simulink model "commhdlQPSKTxRxLoopback"  (R2025b)
settings: Solver=FixedStepDiscrete  StartTime=0.0  StopTime=stopTime  RelTol=1e-3
PostLoadFcn:
  | hScopeConfig = get_param([gcs '/Receiver/QPSK Rx/Frequency and Time Synchronizer/Symbol Synchronizer/No HDL/QPSK Receiver Eye Diagram'],'ScopeConfiguration');
  | 
  | hScopeConfig.OpenAtSimulationStart = false;
  | hScopeConfig.Visible = false;
  | SamplesPerSymbol = 4;
  | %UpsamplesRx = 1;
  | clear hScopeConfig
InitFcn:
  | commhdlQPSKTxRxModelInit;
  | % Rate bridge: ADRV9002/Jupiter radio runs at 15.36 MHz = 2x the 7.68 MHz
  | % (4 samples/symbol @ Rsym=1.92 MHz) the QPSK Rx requires. The deployed
  | % Receiver must downsample the ADC stream by 2. UpsamplesRx=1 fed the QPSK
  | % Rx 8 sps (2x-upsampled) and broke symbol sync / the loopback bit check.
  | UpsamplesRx = 1;   %% T8 RATE FIX: rail 15.36e6 == ADC bus rate,
  | %% no ingress decimation (was 2 when the rail sat on the 7.68e6 rung)
  | UpsamplesTx = 1;
  | clear simTimingOffset;
StopFcn:
  | if exist('simTimingOffset','var')
  |   disp('Simulation completed');
  |   %QPSKTxRxVerification;
  | end
undefined symbols (not defined in the file or in its folder): Add, Config, fsym, randsrc, RandStream, Rsym, Shift
libraries: hdlsllib x141, simulink x43, dspsigops x34, dsphdlfiltering2 x6, dsphdlsigops2 x4, dsphdlmathfun2 x4, commdigbbndpm3 x4, dspmlti4 x2, commchan3 x1, commrflib2 x1, commcnvcod2 x1
(part 1 of 8)
CloseFcn:
  | clear Config CSLatency dataBits dataIn DBPP DescramblerLatency endLoc ...
  |         errSym errWaveform falsePacketsNo FCLatency idx initFramesNotToCompareInRx ...
  |         Nframes nReceivedBits PALatency PDLatency pktNo QPSKDemodLatency ...
  |         refQPSKSym refTxWaveform Rsym RxBits RxOut RxOutEnd RxOutSrt ...
  |         simAfterCS simBeforeSS simPeakFind simQPSKSym simSyncedPackets ...
  |         simTimingOffset simTxWaveform srtLoc SSLatency stopTime tout trueOffset ...
  |         TxBits validIn vPktNo
  | clear SamplesPerSymbol nErrBits nErrPkts nMissedPkts TxSymbolsMaxError TxWaveformMaxError
Description:
  | frame=f1536 variant=jupiter_240k5_byte(sps4/Rsym3840000-T8ratefix,K5[35 23]TB25 rx+GATED-txenc,ROMf1536+byteDMA,noscr+nodescr,taps 0x150/0x154/0x15C,agcEn10,txds 0x158,WPP191) pre=variant_pre_composite_verif+cfc_a12+bytek5 build=12-Aug-2026 10:18:16
settings Model: DataTypeOverride=Off  Creator=The MathWorks, Inc.  LastModifiedBy=tcollins
settings SolverCC: AlgebraicLoopSolver=TrustRegion  MaxZcPerStep=1.0
settings DataIOCC: ReturnWorkspaceOutputs=off
settings OptimizationCC: BlockReduction=off  ConditionallyExecuteInputs=off  DefaultParameterBehavior=Inlined  ReuseModelBlockBuffer=off
settings DebuggingCC: AlgebraicLoopMsg=error  SingleTaskRateTransMsg=error  UnconnectedInputMsg=warning  UnconnectedOutputMsg=warning  UnconnectedLineMsg=warning  SubsystemReferenceDiagnosticForUnitTest=warning
settings HardwareCC: ProdBitPerPointer=32.0  ProdBitPerSizeT=32.0  ProdBitPerPtrDiffT=32.0  ProdLargestAtomicFloat=None  ProdIntDivRoundTo=Undefined  ProdEndianess=Unspecified  ProdWordSize=32.0  ProdHWDeviceType=ASIC/FPGA->ASIC/FPGA  TargetBitPerLong=64.0  TargetBitPerPointer=64.0  TargetBitPerSizeT=64.0  TargetBitPerPtrDiffT=64.0  TargetLongLongMode=on  TargetIntDivRoundTo=Zero  TargetEndianess=LittleEndian  TargetWordSize=64.0  TargetHWDeviceType=Custom Processor->MATLAB Host Computer  ProdEqTarget=off
settings ModelReferenceCC: EnableRefExpFcnMdlSchedulingChecks=on
settings RTWCC: GPUComputeCapability=3.5  DLArmComputeVersion=19.05

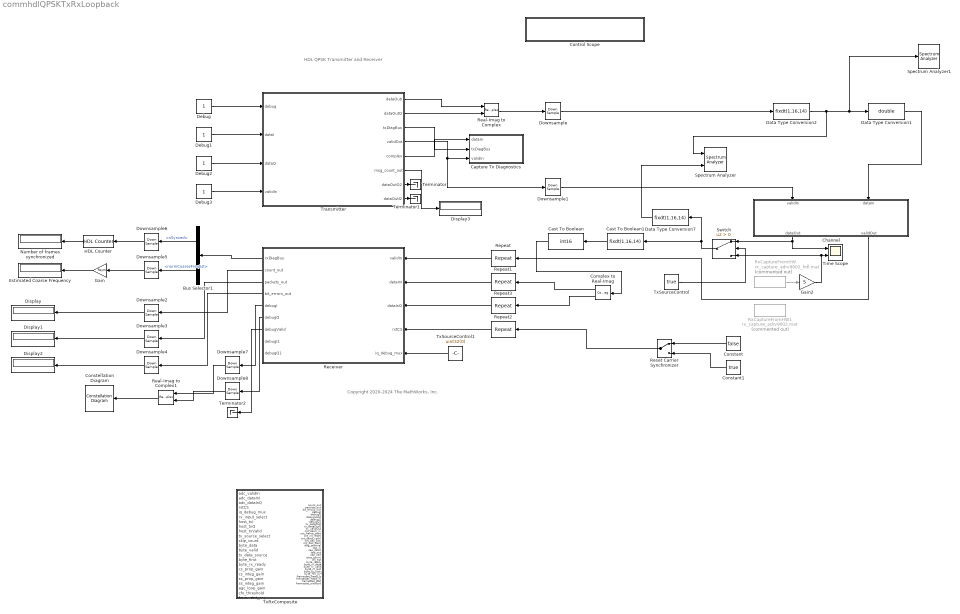
== system commhdlQPSKTxRxLoopback ==
  note: HDL QPSK Transmitter and Receiver
  note: Copyright 2020-2024 The MathWorks, Inc.
  Bus Selector1 : BusSelector  OutputSignals=nSynced,normCoarseFreqEst
  Capture Tx Diagnostics : Subsystem
  Cast To Boolean : DataTypeConversion  OutDataTypeStr=int16  ConvertRealWorld=Stored Integer (SI)  SaturateOnIntegerOverflow=off  RndMeth=Floor
  Cast To Boolean1 : DataTypeConversion  OutDataTypeStr=fixdt(1,16,14)  SaturateOnIntegerOverflow=off  RndMeth=Floor
  Channel : Subsystem  mask{EbN0dB=40, CFO=1e3, CPO=135, fractionalTimingOffset=0.55, timingFrequencyOffset=2}
      mask prompts: EbN0dB "Eb/N0 (in dB) :"; CFO "Carrier Frequency Offset (in Hz):"; CPO "Carrier Phase Offset (in Degrees) :"; fractionalTimingOffset "Fractional Timing Offset ( <1 ) :"; timingFrequencyOffset "Timing Frequency Offset (in PPM) :"
      mask init:
      | validateattributes(fractionalTimingOffset,{'double'},{'finite','scalar','nonnegative','>=',0,'<',1},'','fractionalTimingOffset');
      | validateattributes(timingFrequencyOffset,{'double'},{'finite','scalar','nonnegative'},'','timingFrequencyOffset');
      | validateattributes(EbN0dB,{'double'},{'scalar'},'','EbN0dB');
      | validateattributes(CFO,{'double'},{'finite','scalar',},'','CFO');
      | validateattributes(CPO,{'double'},{'finite','scalar'},'','CPO');
      | 
      | BitsPerSymbol = 2;      % QPSK
      | EbN0          = 10^(EbN0dB/10);
      | EsN0          = BitsPerSymbol*EbN0;
      | noiseVariance = 1/EsN0;  % QPSK symbol energy is normalized to 1 i.e. Es = 1
      | 
      | clear BitsPersymbol EbN0 EsN0
      settings: PortSchema="{\"entries\":[{\"content\":{\"sides\":[{\"content\":{\"connectorIds\":[]},\"type\":\"ConnectorPlacement.EquallySpacedRectSide\",\"uuid\":\"aa9ac445-3d73-401b-8e6c-a43fa6f53e3e\"},{\"content\":{\"connectorIds\":[],\"side\":\"RIGHT\"},\"type\":\"ConnectorPlacement.EquallySpacedRectSide\",\"uuid\":\"c8fbe2c1-ad18-4b81-8824-4fece19db9b5\"},{\"content\":{\"connectorIds\":[\"In1\",\"In2\"],\"side\":\"TOP\"},\"type\":\"ConnectorPlacement.EquallySpacedRectSide\",\"uuid\":\"2fdd8701-02b7-4a19-ab6e-54d2593732fa\"},{\"content\":{\"connectorIds\":[\"Out1\",\"Out2\"],\"side\":\"BOTTOM\"},\"type\":\"ConnectorPlacement.EquallySpacedRectSide\",\"uuid\":\"bd6ca111-71ba-47de-a918-1bcd41b09175\"}]},\"type\":\"ConnectorPlacement.EquallySpacedConnector\",\"uuid\":\"c410269f-5de3-4a8f-bc07-850237ff35fb\"}],\"packageUris\":[\"http://schema.mathworks.com/mf0/Connector/R2020b\"],\"version\":\"1.0\"}"
      mask DialogControl DescGroupVar Prompt: Channel
      mask Display: disp(['Double-Click' newline 'to set channel']);
  Complex to Real-Imag : ComplexToRealImag
  Constant : Constant  Value=false  SampleTime=1/(Rsym*Config.SamplesPerSymbol)
  Constant1 : Constant  Value=true  SampleTime=1/(Rsym*Config.SamplesPerSymbol)
  Constellation Diagram : ConstellationDiagram  WindowPosition=[594.000000,164.000000,600.000000,600.000000,]  Visible=on  ScopeFrameLocation=window  SymbolsToDisplaySource=Property  SymbolsToDisplay=1000  XLimits=[-1.375,8542.5]  YLimits=[-1.375,8542.5]  AxesLimits=[-1.375,8542.5]  MaximizeAxes=on  DefaultConfigurationName=comm.scopes.ConstellationDiagramBlockCfg
  Control Scope : Subsystem
      settings: OpenFcn=|
      | hScopeConfig1 = get_param([gcs '/Capture Tx Diagnostics/QPSK Transmitter Constellations'],'ScopeConfiguration');
      | hScopeConfig2 = get_param([gcs '/QPSK Rx/Frequency and Time Synchronizer/Symbol Synchronizer/No HDL/QPSK Receiver Eye Diagram'],'ScopeConfiguration');
      | hScopeConfig3 = get_param([gcs '/QPSK Rx/Frequency and Time Synchronizer/Symbol Synchronizer/No HDL/No HDL/QPSK Receiver Constellation 1'],'ScopeConfiguration');
      | hScopeConfig4 = get_param([gcs '/QPSK Rx/Frequency and Time Synchronizer/No HDL/QPSK Receiver Constellations 2'],'ScopeConfiguration');
      | hScopeConfig5 = get_param([gcs '/QPSK Rx/Frequency and Time Synchronizer/Preamble Detector/No HDL/Correlation Time Scope'],'ScopeConfiguration');
      | 
      | 
      | 
      | if all([hScopeConfig1.Visible hScopeConfig2.Visible hScopeConfig3.Visible hScopeConfig4.Visible hScopeConfig5.Visible])
      |    hScopeConfig1.Visible = false;
      |    hScopeConfig2.Visible = false;
      |    hScopeConfig3.Visible = false;
      |    hScopeConfig4.Visible = false;
      |    hScopeConfig5.Visible = false;
      | else
      |    hScopeConfig1.Visible = true;
      |    hScopeConfig2.Visible = true;
      |    hScopeConfig3.Visible = true;
      |    hScopeConfig4.Visible = true;
      |    hScopeConfig5.Visible = true;
      | end
      | 
      | clear hScopeConfig1 hScopeConfig2 hScopeConfig3 hScopeConfig4 hScopeConfig5;
      mask Display: disp('Double-click to turn on/off the Scopes');
  Data Type Conversion1 : DataTypeConversion  OutDataTypeStr=double  SaturateOnIntegerOverflow=off  RndMeth=Floor
  Data Type Conversion2 : DataTypeConversion  OutDataTypeStr=fixdt(1,16,14)  ConvertRealWorld=Stored Integer (SI)  SaturateOnIntegerOverflow=off  RndMeth=Floor
  Data Type Conversion7 : DataTypeConversion  OutDataTypeStr=fixdt(1,16,14)  SaturateOnIntegerOverflow=off  RndMeth=Floor
  Debug : Constant  OutDataTypeStr=uint32  SampleTime=-1
  Debug1 : Constant  OutDataTypeStr=int16  SampleTime=-1
  Debug2 : Constant  OutDataTypeStr=int16  SampleTime=-1
  Debug3 : Constant  OutDataTypeStr=boolean  SampleTime=-1
  Display{,1..3} (4 alike) : Display
  Downsample : DownSample  N=UpsamplesTx  RateOptions=Allow multirate processing
  Downsample1 : DownSample  N=UpsamplesTx  RateOptions=Allow multirate processing
  Downsample{2..8} (7 alike) : DownSample  N=UpsamplesRx  RateOptions=Allow multirate processing
  Estimated Coarse Frequency : Display
  Gain : Gain  Gain=Rsym
  Gain2 : Gain  Gain=5
  HDL Counter : hdlsllib/Sources/HDL Counter  CountType=Free running  CountInit=0  CountStep=1  CountMax=25  CountFromType=Initial value  CountFrom=0  CountResetPort=off  CountLoadPort=off  CountEnbPort=on  CountDirPort=off  CountHitOutputPort=off  CountDataType=Unsigned  CountWordLen=32  CountFracLen=0  CountSampTime=1
  Number of frames synchronized : Display
  Real-Imag to Complex : RealImagToComplex
  Real-Imag to Complex1 : RealImagToComplex
  Receiver : Subsystem  TreatAsAtomicUnit=on
  Repeat{,1..3} (4 alike) : dspsigops/Repeat  FactorSource=Dialog parameter  N=UpsamplesRx  Nmax=16  InputProcessing=Columns as channels (frame based)  RateOptions=Allow multirate processing  ic=0  mode=Unused parameter value
      settings: LibrarySourceBlock=commsequence2/Repeat
  Reset Carrier Synchronizer : ManualSwitch
  RxCaptureFromHW : FromFile  Commented=on  FileName=rx_capture_adrv9002_hdl.mat  OutDataTypeStr=double  SampleTime=1/(Rsym*Config.SamplesPerSymbol)  ExtrapolationBeforeFirstDataPoint=Hold first value  InterpolationWithinTimeRange=Zero order hold  ExtrapolationAfterLastDataPoint=Hold last value
  RxCaptureFromHW1 : FromFile  Commented=on  FileName=rx_capture_adrv9002.mat  OutDataTypeStr=double  SampleTime=1/(Rsym*Config.SamplesPerSymbol)  ExtrapolationBeforeFirstDataPoint=Hold first value  InterpolationWithinTimeRange=Zero order hold  ExtrapolationAfterLastDataPoint=Hold last value
  Spectrum Analyzer : SpectrumAnalyzer  NumInputPorts=2  WindowPosition=[494.000000,214.000000,800.000000,500.000000,]  Visible=on  ScopeFrameLocation=window  WindowInvariantSamplesPerUpdate=on  Span=7680000  StartFrequency=-3840000  StopFrequency=3840000  YLimits=[-47.9968 8.4452]
  Spectrum Analyzer1 : SpectrumAnalyzer  WindowPosition=[494.000000,214.000000,800.000000,500.000000,]  Visible=on  ScopeFrameLocation=window  WindowInvariantSamplesPerUpdate=on  Span=7680000  StartFrequency=-3840000  StopFrequency=3840000  YLimits=[-71.5508 10.9276]
  Switch : Switch  Criteria=u2 > Threshold  SaturateOnIntegerOverflow=off  InputSameDT=off
  Terminator : Terminator
  Terminator1 : Terminator
  Terminator2 : Terminator
  Time Scope : Scope  NumInputPorts=2
      settings: TimeUnits=Metric (based on Time Span)  ActiveDisplayYMinimum=-1.0052287666621835  ActiveDisplayYMaximum=0.87958747263253323  YLabel=Amplitude
  Transmitter : Subsystem  TreatAsAtomicUnit=on
  TxRxComposite : Subsystem
  TxSourceControl : Constant  Value=true  SampleTime=-1
  TxSourceControl1 : Constant  Value=uint32(0)  SampleTime=-1
  wires:
  Bus Selector1/1 -> Downsample6/1  "<nSynced>"
  HDL Counter/1 -> Number of frames synchronized/1
  Bus Selector1/2 -> Downsample5/1  "<normCoarseFreqEst>"
  Gain/1 -> Estimated Coarse Frequency/1
  Data Type Conversion1/1 -> Channel/2(dataIn)
  Constant/1 -> Reset Carrier Synchronizer/1
  Constant1/1 -> Reset Carrier Synchronizer/2
  Channel/1(dataOut) -> Time Scope/1, Switch/1
  Switch/1 -> Data Type Conversion7/1, Cast To Boolean1/1
  TxSourceControl/1 -> Switch/2
  RxCaptureFromHW/1 -> Gain2/1
  Gain2/1 -> Switch/3, Time Scope/2
  Transmitter/4(validOut) -> Downsample1/1, Capture Tx Diagnostics/3(validIn)
  Transmitter/3(txDiagBus) -> Capture Tx Diagnostics/2(txDiagBus)
  Debug/1 -> Transmitter/1(debug)
  Channel/2(validOut) -> Repeat/1
  Reset Carrier Synchronizer/1 -> Repeat2/1
  Receiver/2(count_out) -> Downsample2/1
  Receiver/3(packets_out) -> Downsample3/1
  Receiver/4(bit_errors_out) -> Downsample4/1
  Debug2/1 -> Transmitter/3(dataQ)
  Debug1/1 -> Transmitter/2(dataI)
  Debug3/1 -> Transmitter/4(validIn)
  Transmitter/1(dataOutI) -> Real-Imag to Complex/1
  Transmitter/2(dataOutQ) -> Real-Imag to Complex/2
  Real-Imag to Complex/1 -> Downsample/1
  Transmitter/5(complex) -> Capture Tx Diagnostics/1(dataIn)
  Data Type Conversion2/1 -> Spectrum Analyzer/1, Spectrum Analyzer1/1, Data Type Conversion1/1
  Transmitter/6(msg_count_out) -> Display3/1
  Downsample/1 -> Data Type Conversion2/1
  Downsample1/1 -> Channel/1(validIn)
  Repeat/1 -> Receiver/1(validIn)
  Repeat1/1 -> Receiver/2(dataInI)
  Repeat2/1 -> Receiver/4(rstCS)
  Downsample2/1 -> Display/1
  Downsample3/1 -> Display1/1
  Downsample4/1 -> Display2/1
  Receiver/1(rxDiagBus) -> Bus Selector1/1
  Downsample5/1 -> Gain/1
  Downsample6/1 -> HDL Counter/1
  Transmitter/7(dataOutQ2) -> Terminator/1
  Transmitter/8(dataOutI2) -> Terminator1/1
  TxSourceControl1/1 -> Receiver/5(iq_debug_mux)
  Complex to Real-Imag/1 -> Repeat1/1
  Complex to Real-Imag/2 -> Repeat3/1
  Data Type Conversion7/1 -> Spectrum Analyzer/2
  Cast To Boolean/1 -> Complex to Real-Imag/1
  Repeat3/1 -> Receiver/3(dataInQ)
  Cast To Boolean1/1 -> Cast To Boolean/1
  Receiver/5(debugI) -> Downsample7/1
  Receiver/6(debugQ) -> Downsample8/1
  Downsample7/1 -> Real-Imag to Complex1/1
  Downsample8/1 -> Real-Imag to Complex1/2
  Real-Imag to Complex1/1 -> Constellation Diagram/1
  Receiver/7(debugValid) -> Terminator2/1

== system commhdlQPSKTxRxLoopback/Capture Tx Diagnostics ==
  dataIn : Inport
  txDiagBus : Inport  Port=2
  validIn : Inport  Port=3
  Bus Selector : BusSelector  OutputSignals=QPSKConstellationPoints,QPSKConstellationValid
  Data Type Conversion : DataTypeConversion  OutDataTypeStr=double  SaturateOnIntegerOverflow=off  RndMeth=Floor
  Data Type Conversion1 : DataTypeConversion  OutDataTypeStr=double  SaturateOnIntegerOverflow=off  RndMeth=Floor
  QPSK Transmitter Constellations : ConstellationDiagram  NumInputPorts=2  WindowPosition=[708.000000,285.000000,372.000000,357.000000,]  Visible=on  ScopeFrameLocation=window  SymbolsToDisplaySource=Property  SymbolsToDisplay=10000  ReferenceConstellation="{[0.70711+0.70711i        -0.70711+0.70711i        -0.70711-0.70711i         0.70711-0.70711i],[0.70711+0.70711i        -0.70711+0.70711i        -0.70711-0.70711i         0.70711-0.70711i]}"  ReferenceMarker={''o'',''o''}  ReferenceColor={[1 0 0],[1 0 0]}  XLimits=[-0.94638 0.94638]  YLimits=[-0.94638 0.94638]  AxesLimits=[-0.94638 0.94638]  ShowLegend=on  DefaultConfigurationName=comm.scopes.ConstellationDiagramBlockCfg
      settings: OpenAtSimulationStart=off
  Subsystem : Subsystem
  Subsystem1 : Subsystem
  Unit Delay Enabled Synchronous : hdlsllib/Discrete/Unit Delay Enabled Synchronous  InitialCondition=0.0  SampleTime=-1
  Unit Delay Enabled Synchronous1 : hdlsllib/Discrete/Unit Delay Enabled Synchronous  InitialCondition=0.0  SampleTime=-1
  wires:
  txDiagBus/1 -> Bus Selector/1
  Bus Selector/1 -> Data Type Conversion/1  "<QPSKConstellationPoints>"
  Data Type Conversion/1 -> Unit Delay Enabled Synchronous/1, Subsystem/1(In1)
  dataIn/1 -> Data Type Conversion1/1
  Bus Selector/2 -> Subsystem/Enable, Unit Delay Enabled Synchronous/2  "<QPSKConstellationValid>"
  Data Type Conversion1/1 -> Unit Delay Enabled Synchronous1/1, Subsystem1/1(In1)
  validIn/1 -> Subsystem1/Enable, Unit Delay Enabled Synchronous1/2
  Unit Delay Enabled Synchronous1/1 -> QPSK Transmitter Constellations/2  "RRC Filtered Output"
  Unit Delay Enabled Synchronous/1 -> QPSK Transmitter Constellations/1  "Modulator Output"

== system commhdlQPSKTxRxLoopback/Channel ==
  validIn : Inport
  dataIn : Inport  Port=2
  AWGN Channel : commchan3/AWGN Channel  LegacyMode=on  NoiseMethod="Signal to noise ratio  (SNR)"  noiseMode=Variance from mask  EbNo=EbN0dB  EsNo=10  SNR=10  BitsPerSymbol=2  SignalPower=1  SpecifySymbolPeriod=off  SamplesPerSymbol=1  SymbolPeriod=1/fsym  VarianceSource=Parameter  Variance=noiseVariance  RandomStream=Global stream  Seed=67  SimulateUsing=Code generation
  Add : Sum  Inputs=|++
  Add1 : Sum  Inputs=++|
  Constant : Constant  Value=fractionalTimingOffset  SampleTime=-1
  Constant1 : Constant  Value=timingFrequencyOffset * 1e-6  SampleTime=-1
  Delay : Delay  DelayLength=1
  Mod 1 : Subsystem
  Phase/ Frequency Offset : commrflib2/Phase// Frequency Offset  phaseOffset=CPO  freqPort=off  freqOffset=CFO
  Variable Fractional Delay : dspsigops/Variable Fractional Delay  mode=OBSOLETE  modeActive=Linear  L=4  FarrowL=4  R=10  alpha=1  dmax=100  InputProcessing=Columns as channels (frame based)  ic=0  noDFT=off  fallbackFIR=Clip to the minimum value necessary for centered kernel  fallbackFarrow=Clip to the minimum value necessary for centered kernel  roundingMode=Zero  overflowMode=off
  dataOut : Outport
  validOut : Outport  Port=2
  wires:
  AWGN Channel/1 -> Phase/ Frequency Offset/1
  Variable Fractional Delay/1 -> AWGN Channel/1
  dataIn/1 -> Variable Fractional Delay/1
  Constant1/1 -> Add/1
  Delay/1 -> Add/2, Add1/2
  Add/1 -> Delay/1
  Add1/1 -> Mod 1/1(In1)
  Constant/1 -> Add1/1
  Mod 1/1(Out1) -> Variable Fractional Delay/2
  Phase/ Frequency Offset/1 -> dataOut/1
  validIn/1 -> validOut/1

== system commhdlQPSKTxRxLoopback/Control Scope ==

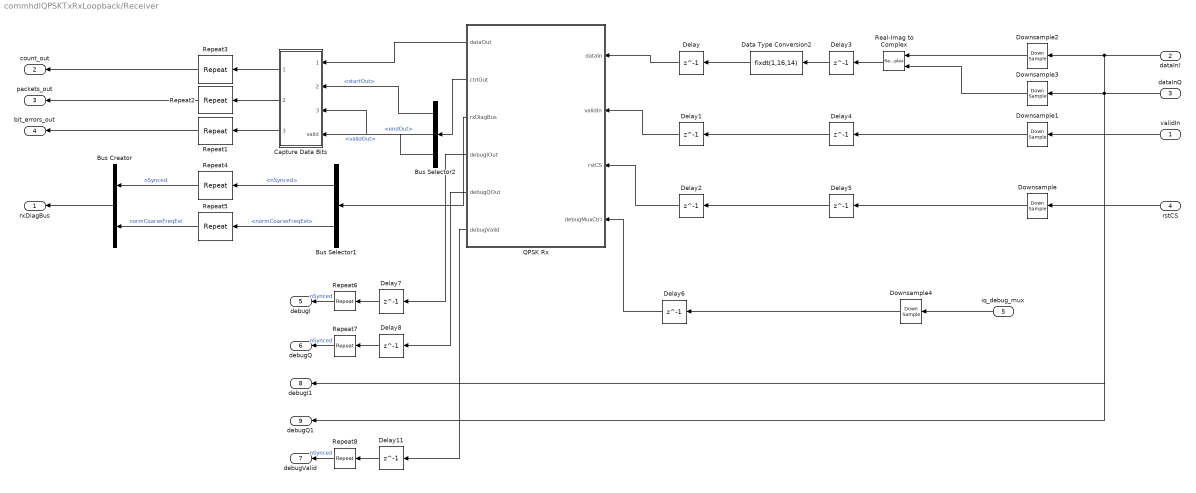
== system commhdlQPSKTxRxLoopback/Receiver ==
  validIn : Inport
  dataInI : Inport  Port=2
  dataInQ : Inport  Port=3
  rstCS : Inport  Port=4
  iq_debug_mux : Inport  Port=5  OutDataTypeStr=uint32
  Bus Creator : BusCreator  Inputs=2
  Bus Selector1 : BusSelector  OutputSignals=nSynced,normCoarseFreqEst
  Bus Selector2 : BusSelector  OutputSignals=startOut,endOut,validOut
  Capture Data Bits : Subsystem
  Data Type Conversion2 : DataTypeConversion  OutDataTypeStr=fixdt(1,16,14)  ConvertRealWorld=Stored Integer (SI)  SaturateOnIntegerOverflow=off  RndMeth=Floor
  Delay{,1..8,11} (10 alike) : Delay  DelayLength=1
  Downsample{,1..4} (5 alike) : DownSample  N=UpsamplesRx  RateOptions=Allow multirate processing
  QPSK Rx : Subsystem
      mask init:
      | integAvgLen = 2^12;
      | 
      | RxParams            = commhdlQPSKTxRxParameters();
      | Preamble            = RxParams.Preamble;
      | QPSKConstellation   = RxParams.QPSKConstellation;
      | dataBitsPerPacket   = RxParams.DataBitsPerPacket;
      | SamplesPerSymbol    = RxParams.SamplesPerSymbol;
      | RRCCoef             = RxParams.RRCCoef;
      | bitsPerPacket        = RxParams.BitsPerPacket;
      | 
      | rxPreambleMFCoeffs  = RxParams.rxPreambleMFCoeffs;
      | preambleSymbols     = RxParams.preambleSymbols;
      | ThresoldGainFac     = RxParams.ThresoldGainFac;
      | 
      | % AGC Parameters
      | AGCReference           = RxParams.AGCReference;
      | AGCLoopGain            = RxParams.AGCLoopGain;
      | 
      | % CS parameters
      | CSKp                   = RxParams.CSKp;
      | CSK0                   = RxParams.CSK0;  
      | CSLoopFilterPropGain   = RxParams.CSLoopFilterPropGain;
      | CSLoopFilterIntegGain  = RxParams.CSLoopFilterIntegGain;
      | CFOChangeDetectThreshold = RxParams.CFOChangeDetectThreshold;
      | 
      | % SS parameters
      | SSKp                   = RxParams.SSKp; 
      | SSK0                   = RxParams.SSK0;  
      | SSLoopFilterPropGain   = RxParams.SSLoopFilterPropGain;
      | SSLoopFilterIntegGain  = RxParams.SSLoopFilterIntegGain;
      | 
      | % preamble detector parameters
      | searchSamples          = RxParams.SearchSamples;
      | 
      | clear RxParams;
  Real-Imag to Complex : RealImagToComplex
  Repeat{1..8} (8 alike) : dspsigops/Repeat  FactorSource=Dialog parameter  N=UpsamplesRx  Nmax=16  InputProcessing=Columns as channels (frame based)  RateOptions=Allow multirate processing  ic=0  mode=Unused parameter value
      settings: LibrarySourceBlock=commsequence2/Repeat
  rxDiagBus : Outport
  count_out : Outport  Port=2
  packets_out : Outport  Port=3
  bit_errors_out : Outport  Port=4
  debugI : Outport  Port=5
  debugQ : Outport  Port=6
  debugValid : Outport  Port=7
  debugI1 : Outport  Port=8
  debugQ1 : Outport  Port=9
  wires:
  Bus Selector2/1 -> Capture Data Bits/2(dataSrt)  "<startOut>"
  QPSK Rx/1(dataOut) -> Capture Data Bits/1(dataOut)
  QPSK Rx/2(ctrlOut) -> Bus Selector2/1
  Bus Selector2/2 -> Capture Data Bits/3(dataEnd)  "<endOut>"
  rstCS/1 -> Downsample/1
  validIn/1 -> Downsample1/1
  Bus Selector2/3 -> Capture Data Bits/4(valid)  "<validOut>"
  Capture Data Bits/1(count_out) -> Repeat3/1
  Capture Data Bits/2(packets_out) -> Repeat2/1
  Capture Data Bits/3(bit_errors_out) -> Repeat1/1
  Downsample1/1 -> Delay4/1
  Repeat1/1 -> bit_errors_out/1
  Repeat2/1 -> packets_out/1
  Repeat3/1 -> count_out/1
  QPSK Rx/3(rxDiagBus) -> Bus Selector1/1
  Bus Creator/1 -> rxDiagBus/1
  Bus Selector1/1 -> Repeat4/1  "<nSynced>"
  Bus Selector1/2 -> Repeat5/1  "<normCoarseFreqEst>"
  Repeat4/1 -> Bus Creator/1  "nSynced"
  Repeat5/1 -> Bus Creator/2  "normCoarseFreqEst"
  dataInQ/1 -> debugQ1/1, Downsample3/1
  dataInI/1 -> debugI1/1, Downsample2/1
  Real-Imag to Complex/1 -> Delay3/1
  Downsample2/1 -> Real-Imag to Complex/1
  Downsample3/1 -> Real-Imag to Complex/2
  Data Type Conversion2/1 -> Delay/1
  Delay/1 -> QPSK Rx/1(dataIn)
  Delay1/1 -> QPSK Rx/2(validIn)
  Delay2/1 -> QPSK Rx/3(rstCS)
  Delay3/1 -> Data Type Conversion2/1
  Delay4/1 -> Delay1/1
  Delay5/1 -> Delay2/1
  QPSK Rx/4(debugIOut) -> Delay7/1
  QPSK Rx/5(debugQOut) -> Delay8/1
  Repeat6/1 -> debugI/1  "nSynced"
  Repeat7/1 -> debugQ/1  "nSynced"
  iq_debug_mux/1 -> Downsample4/1
  Delay6/1 -> QPSK Rx/4(debugMuxCtrl)
  Downsample4/1 -> Delay6/1
  Repeat8/1 -> debugValid/1  "nSynced"
  QPSK Rx/6(debugValid) -> Delay11/1
  Delay7/1 -> Repeat6/1
  Delay8/1 -> Repeat7/1
  Delay11/1 -> Repeat8/1
  Downsample/1 -> Delay5/1

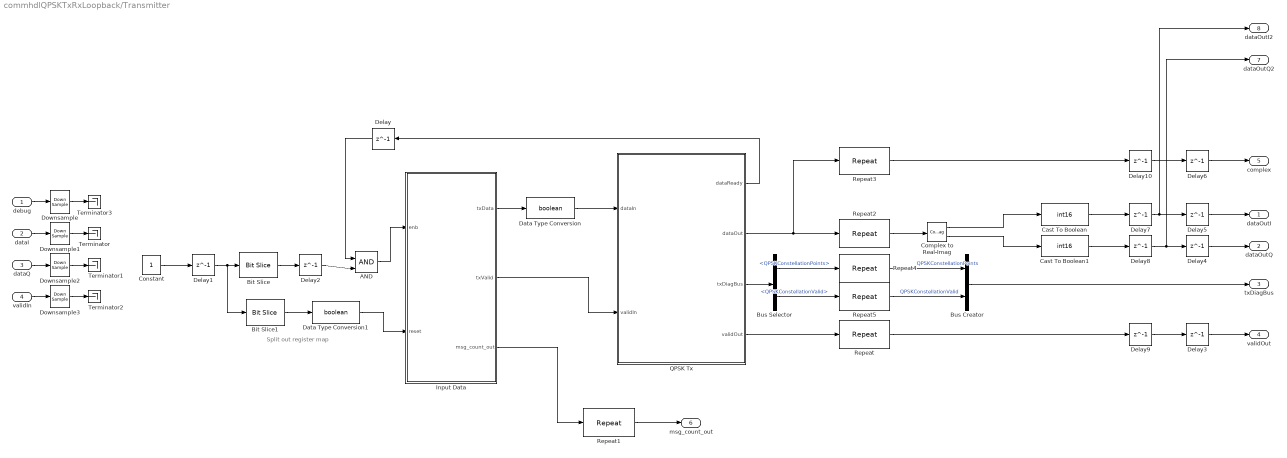
== system commhdlQPSKTxRxLoopback/Transmitter ==
  note: Split out register map
  debug : Inport  PortDimensions=1
  dataI : Inport  Port=2
  dataQ : Inport  Port=3
  validIn : Inport  Port=4
  AND : Logic  IconShape=distinctive  AllPortsSameDT=off  OutDataTypeStr=boolean
  Bit Slice : hdlsllib/Logic and Bit Operations/Bit Slice  lidx=0  ridx=0
  Bit Slice1 : hdlsllib/Logic and Bit Operations/Bit Slice  lidx=1  ridx=1
  Bus Creator : BusCreator  Inputs=2
  Bus Selector : BusSelector  OutputSignals=QPSKConstellationPoints,QPSKConstellationValid
  Cast To Boolean : DataTypeConversion  OutDataTypeStr=int16  ConvertRealWorld=Stored Integer (SI)  SaturateOnIntegerOverflow=off  RndMeth=Floor
  Cast To Boolean1 : DataTypeConversion  OutDataTypeStr=int16  ConvertRealWorld=Stored Integer (SI)  SaturateOnIntegerOverflow=off  RndMeth=Floor
  Complex to Real-Imag : ComplexToRealImag
  Constant : Constant  OutDataTypeStr=uint32  SampleTime=-1
  Data Type Conversion : DataTypeConversion  OutDataTypeStr=boolean  SaturateOnIntegerOverflow=off  RndMeth=Floor
  Data Type Conversion1 : DataTypeConversion  OutDataTypeStr=boolean  SaturateOnIntegerOverflow=off  RndMeth=Floor
  Delay{,1..10} (11 alike) : Delay  DelayLength=1
  Downsample{,1..3} (4 alike) : DownSample  N=UpsamplesTx  RateOptions=Allow multirate processing
  Input Data : Subsystem  mask{dataBits=reshape(repmat(randsrc(2240*1,1,[0,1],RandStream('mcg16807','Seed',0)), 59,1), [2240*59,1]), Rsym=3.84e6}
      mask prompts: dataBits "Data Bits :"; Rsym "Symbol Rate (in baud rate)  :"
      mask Display: disp(['Double-Click' newline 'to set data bits']);
  QPSK Tx : Subsystem
      mask init:
      | TxParams           = commhdlQPSKTxRxParameters();
      | Preamble            = TxParams.Preamble;
      | QPSKConstellation   = TxParams.QPSKConstellation;
      | dataBitsPerPacket   = TxParams.DataBitsPerPacket;
      | SamplesPerSymbol    = TxParams.SamplesPerSymbol;
      | RRCCoef             = TxParams.RRCCoef;
      | dataRAMAddrWidth    = TxParams.txDataRAMAddrWidth;
      | bitsPerPacket       = TxParams.BitsPerPacket;
      | 
      | clear TxParams;
  Repeat{,1..5} (6 alike) : dspsigops/Repeat  FactorSource=Dialog parameter  N=UpsamplesTx  Nmax=16  InputProcessing=Columns as channels (frame based)  RateOptions=Allow multirate processing  ic=0  mode=Unused parameter value
      settings: LibrarySourceBlock=commsequence2/Repeat
  Terminator{,1..3} (4 alike) : Terminator
  dataOutI : Outport
  dataOutQ : Outport  Port=2
  txDiagBus : Outport  Port=3
  validOut : Outport  Port=4
  complex : Outport  Port=5
  msg_count_out : Outport  Port=6
  dataOutQ2 : Outport  Port=7
  dataOutI2 : Outport  Port=8
  wires:
  Input Data/2(txValid) -> QPSK Tx/2(validIn)
  Input Data/1(txData) -> Data Type Conversion/1
  Data Type Conversion/1 -> QPSK Tx/1(dataIn)
  QPSK Tx/4(validOut) -> Repeat/1
  QPSK Tx/1(dataReady) -> Delay/1
  AND/1 -> Input Data/1(enb)
  Bit Slice/1 -> Delay2/1
  Delay/1 -> AND/1
  Delay1/1 -> Bit Slice1/1, Bit Slice/1
  Delay2/1 -> AND/2
  Bit Slice1/1 -> Data Type Conversion1/1
  Data Type Conversion1/1 -> Input Data/2(reset)
  dataI/1 -> Downsample1/1
  dataQ/1 -> Downsample2/1
  validIn/1 -> Downsample3/1
  Constant/1 -> Delay1/1
  debug/1 -> Downsample/1
  QPSK Tx/2(dataOut) -> Repeat3/1, Repeat2/1
  Complex to Real-Imag/1 -> Cast To Boolean/1
  Complex to Real-Imag/2 -> Cast To Boolean1/1
  Input Data/3(msg_count_out) -> Repeat1/1
  Repeat/1 -> Delay9/1
  Repeat2/1 -> Complex to Real-Imag/1
  Repeat3/1 -> Delay10/1
  Downsample/1 -> Terminator3/1
  Downsample1/1 -> Terminator/1
  Downsample2/1 -> Terminator1/1
  Downsample3/1 -> Terminator2/1
  Repeat1/1 -> msg_count_out/1
  QPSK Tx/3(txDiagBus) -> Bus Selector/1
  Bus Selector/1 -> Repeat4/1  "<QPSKConstellationPoints>"
  Repeat4/1 -> Bus Creator/1  "QPSKConstellationPoints"
  Bus Selector/2 -> Repeat5/1  "<QPSKConstellationValid>"
  Repeat5/1 -> Bus Creator/2  "QPSKConstellationValid"
  Bus Creator/1 -> txDiagBus/1
  Cast To Boolean/1 -> Delay7/1
  Cast To Boolean1/1 -> Delay8/1
  Delay3/1 -> validOut/1
  Delay4/1 -> dataOutQ/1
  Delay5/1 -> dataOutI/1
  Delay6/1 -> complex/1
  Delay7/1 -> dataOutI2/1, Delay5/1
  Delay8/1 -> dataOutQ2/1, Delay4/1
  Delay9/1 -> Delay3/1
  Delay10/1 -> Delay6/1

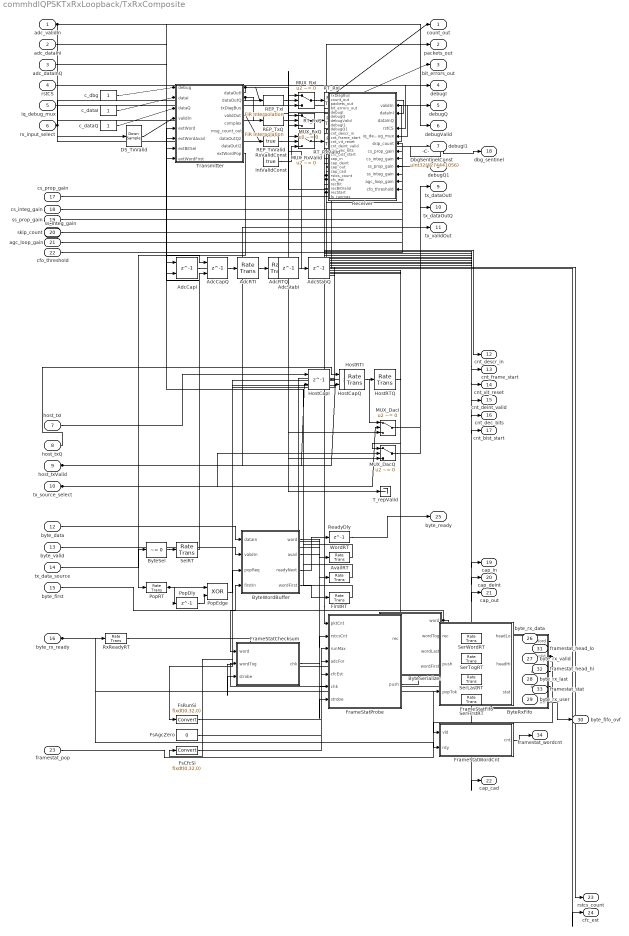
== system commhdlQPSKTxRxLoopback/TxRxComposite ==
  adc_validIn : Inport  OutDataTypeStr=boolean  SampleTime=1/30.72e6
  adc_dataInI : Inport  Port=2  OutDataTypeStr=int16  SampleTime=1/30.72e6
  adc_dataInQ : Inport  Port=3  OutDataTypeStr=int16  SampleTime=1/30.72e6
  rstCS : Inport  Port=4  OutDataTypeStr=boolean  SampleTime=1/15.36e6
  iq_debug_mux : Inport  Port=5  OutDataTypeStr=uint32  SampleTime=1/15.36e6
  rx_input_select : Inport  Port=6  OutDataTypeStr=boolean  SampleTime=1/15.36e6
  host_txI : Inport  Port=7  OutDataTypeStr=int16  SampleTime=1/30.72e6
  host_txQ : Inport  Port=8  OutDataTypeStr=int16  SampleTime=1/30.72e6
  host_txValid : Inport  Port=9  OutDataTypeStr=boolean  SampleTime=1/30.72e6
  tx_source_select : Inport  Port=10  OutDataTypeStr=uint32  SampleTime=1/15.36e6
  skip_count : Inport  Port=11  OutDataTypeStr=uint32  SampleTime=1/15.36e6
  byte_data : Inport  Port=12  OutDataTypeStr=uint64  SampleTime=1/30.72e6
  byte_valid : Inport  Port=13  OutDataTypeStr=boolean  SampleTime=1/30.72e6
  tx_data_source : Inport  Port=14  OutDataTypeStr=uint32  SampleTime=1/15.36e6
  byte_first : Inport  Port=15  OutDataTypeStr=boolean  SampleTime=1/30.72e6
  byte_rx_ready : Inport  Port=16  OutDataTypeStr=boolean  SampleTime=1/30.72e6
  cs_prop_gain : Inport  Port=17  OutDataTypeStr=uint32  SampleTime=1/15.36e6
  cs_integ_gain : Inport  Port=18  OutDataTypeStr=uint32  SampleTime=1/15.36e6
  ss_prop_gain : Inport  Port=19  OutDataTypeStr=uint32  SampleTime=1/15.36e6
  ss_integ_gain : Inport  Port=20  OutDataTypeStr=uint32  SampleTime=1/15.36e6
  agc_loop_gain : Inport  Port=21  OutDataTypeStr=uint32  SampleTime=1/15.36e6
  cfo_threshold : Inport  Port=22  OutDataTypeStr=uint32  SampleTime=1/15.36e6
  framestat_pop : Inport  Port=23  OutDataTypeStr=uint32  SampleTime=1/15.36e6
  AdcCapI : Delay  DelayLength=1  ShowEnablePort=on
      settings: InputPortMap=u0,e6
  AdcCapQ : Delay  DelayLength=1  ShowEnablePort=on
      settings: InputPortMap=u0,e6
  AdcRTI : RateTransition  OutPortSampleTime=1/15.36e6
  AdcRTQ : RateTransition  OutPortSampleTime=1/15.36e6
  AdcStabI : Delay  DelayLength=1
  AdcStabQ : Delay  DelayLength=1
  AvailRT : RateTransition  OutPortSampleTime=1/15.36e6
  ByteRxFifo : MATLAB Function  TreatAsAtomicUnit=on
  ByteSel : simulink/Logic and Bit Operations/Compare To Constant  relop=~=  const=0  OutDataTypeStr=boolean
  ByteSerializer : MATLAB Function  TreatAsAtomicUnit=on
  ByteWordBuffer : MATLAB Function  TreatAsAtomicUnit=on
  DS_TxValid : DownSample  N=1  RateOptions=Allow multirate processing  AllowArbitraryFixedInput=on
  DbgSentinelConst : Constant  Value=uint32(4274441056)  OutDataTypeStr=uint32  SampleTime=1/15.36e6
  FirstRT : RateTransition  OutPortSampleTime=1/15.36e6
  FrameStatChecksum : MATLAB Function  TreatAsAtomicUnit=on
  FrameStatFifo : MATLAB Function  TreatAsAtomicUnit=on
  FrameStatProbe : MATLAB Function  TreatAsAtomicUnit=on
  FrameStatWordCnt : MATLAB Function  TreatAsAtomicUnit=on
  FsAgcZero : Constant  Value=0  OutDataTypeStr=uint32
  FsCfcSi : DataTypeConversion  OutDataTypeStr=fixdt(0,32,0)  ConvertRealWorld=Stored Integer (SI)  SaturateOnIntegerOverflow=off  RndMeth=Floor
  FsRunSi : DataTypeConversion  OutDataTypeStr=fixdt(0,32,0)  ConvertRealWorld=Stored Integer (SI)  SaturateOnIntegerOverflow=off  RndMeth=Floor
  HostCapI : Delay  DelayLength=1  ShowEnablePort=on
      settings: InputPortMap=u0,e6
  HostCapQ : Delay  DelayLength=1  ShowEnablePort=on
      settings: InputPortMap=u0,e6
  HostRTI : RateTransition  OutPortSampleTime=1/30.72e6
  HostRTQ : RateTransition  OutPortSampleTime=1/30.72e6
  IntValidConst : Constant  Value=true  OutDataTypeStr=boolean  SampleTime=1/15.36e6
  MUX_DacI : Switch  Criteria=u2 ~= 0
  MUX_DacQ : Switch  Criteria=u2 ~= 0
  MUX_RxI : Switch  Criteria=u2 ~= 0
  MUX_RxQ : Switch  Criteria=u2 ~= 0
  MUX_RxValid : Switch  Criteria=u2 ~= 0
  PopDly : Delay  DelayLength=1
  PopEdge : Logic  Operator=XOR
  PopRT : RateTransition  OutPortSampleTime=1/30.72e6
  REP_TxI : dspmlti4/FIR Interpolation  FilterSource=Dialog parameters  PrivateCoeffs=0  h=2*fir1(24,0.45)  L=2  FilterObject=FINTERP  framing=Allow multirate processing  outputBufInitCond=0  roundingMode=Nearest  overflowMode=on  firstCoeffDataTypeStr=Inherit: Same word length as input  firstCoeffMin=[]  firstCoeffMax=[]  firstCoeffLastDataTypeStr=Inherit: Same word length as input  outputMin=[]  outputMax=[]
  REP_TxQ : dspmlti4/FIR Interpolation  FilterSource=Dialog parameters  PrivateCoeffs=0  h=2*fir1(24,0.45)  L=2  FilterObject=FINTERP  framing=Allow multirate processing  outputBufInitCond=0  roundingMode=Nearest  overflowMode=on  firstCoeffDataTypeStr=Inherit: Same word length as input  firstCoeffMin=[]  firstCoeffMax=[]  firstCoeffLastDataTypeStr=Inherit: Same word length as input  outputMin=[]  outputMax=[]
  REP_TxValid : dspsigops/Repeat  FactorSource=Dialog parameter  N=2  Nmax=16  RateOptions=Allow multirate processing  ic=0  mode=Unused parameter value
  RT_RxI : RateTransition  OutPortSampleTime=1/15.36e6
  RT_RxQ : RateTransition  OutPortSampleTime=1/15.36e6
  RT_RxValid : RateTransition  OutPortSampleTime=1/15.36e6
  ReadyDly : Delay  DelayLength=1  InitialCondition=1
  Receiver : Subsystem  TreatAsAtomicUnit=on
  RxReadyRT : RateTransition  OutPortSampleTime=1/15.36e6
  RxValidConst : Constant  Value=true  OutDataTypeStr=boolean  SampleTime=1/15.36e6
  SelRT : RateTransition  OutPortSampleTime=1/15.36e6
  SerFirstRT : RateTransition  OutPortSampleTime=1/30.72e6
  SerLastRT : RateTransition  OutPortSampleTime=1/30.72e6
  SerTogRT : RateTransition  OutPortSampleTime=1/30.72e6
  SerWordRT : RateTransition  OutPortSampleTime=1/30.72e6
  T_repValid : Terminator
  Transmitter : Subsystem  TreatAsAtomicUnit=on
  WordRT : RateTransition  OutPortSampleTime=1/15.36e6
  c_dataI : Constant  OutDataTypeStr=int16  SampleTime=1/15.36e6
  c_dataQ : Constant  OutDataTypeStr=int16  SampleTime=1/15.36e6
  c_dbg : Constant  OutDataTypeStr=uint32  SampleTime=1/15.36e6
  count_out : Outport
  packets_out : Outport  Port=2
  bit_errors_out : Outport  Port=3
  debugI : Outport  Port=4
  debugQ : Outport  Port=5
  debugValid : Outport  Port=6
  debugI1 : Outport  Port=7
  debugQ1 : Outport  Port=8
  tx_dataOutI : Outport  Port=9
  tx_dataOutQ : Outport  Port=10
  tx_validOut : Outport  Port=11
  cnt_descr_in : Outport  Port=12
  cnt_frame_start : Outport  Port=13
  cnt_vit_reset : Outport  Port=14
  cnt_deint_valid : Outport  Port=15
  cnt_dec_bits : Outport  Port=16
  cnt_bist_start : Outport  Port=17
  dbg_sentinel : Outport  Port=18
  cap_in : Outport  Port=19
  cap_deint : Outport  Port=20
  cap_out : Outport  Port=21
  cap_cad : Outport  Port=22
  rstcs_count : Outport  Port=23
  cfc_est : Outport  Port=24
  byte_ready : Outport  Port=25
  byte_rx_data : Outport  Port=26
  byte_rx_valid : Outport  Port=27
  byte_rx_last : Outport  Port=28
  byte_rx_user : Outport  Port=29
  byte_fifo_ovf : Outport  Port=30
  framestat_head_lo : Outport  Port=31
  framestat_head_hi : Outport  Port=32
  framestat_stat : Outport  Port=33
  framestat_wordcnt : Outport  Port=34
  wires:
  adc_validIn/1 -> DS_TxValid/1, AdcCapI/2, AdcCapQ/2, debugValid/1
  c_dbg/1 -> Transmitter/1(debug)
  c_dataI/1 -> Transmitter/2(dataI)
  c_dataQ/1 -> Transmitter/3(dataQ)
  DS_TxValid/1 -> Transmitter/4(validIn)
  Transmitter/4(validOut) -> REP_TxValid/1
  rx_input_select/1 -> MUX_RxI/2, MUX_RxQ/2, MUX_RxValid/2
  MUX_RxValid/1 -> RT_RxValid/1
  MUX_RxI/1 -> RT_RxI/1
  MUX_RxQ/1 -> RT_RxQ/1
  RT_RxValid/1 -> Receiver/1(validIn)
  RT_RxI/1 -> Receiver/2(dataInI)
  RT_RxQ/1 -> Receiver/3(dataInQ)
  rstCS/1 -> Receiver/4(rstCS)
  iq_debug_mux/1 -> Receiver/5(iq_debug_mux)
  Receiver/2(count_out) -> count_out/1
  Receiver/3(packets_out) -> packets_out/1, FrameStatProbe/1(pktCnt)
  Receiver/4(bit_errors_out) -> bit_errors_out/1
  Receiver/8(debugI1) -> debugI1/1
  Receiver/9(debugQ1) -> debugQ1/1
  Transmitter/1(dataOutI) -> REP_TxI/1, MUX_RxI/3
  Transmitter/2(dataOutQ) -> REP_TxQ/1, MUX_RxQ/3
  IntValidConst/1 -> MUX_RxValid/3
  host_txI/1 -> HostCapI/1
  host_txValid/1 -> HostCapI/2, HostCapQ/2, tx_validOut/1
  HostCapI/1 -> HostRTI/1
  host_txQ/1 -> HostCapQ/1
  HostCapQ/1 -> HostRTQ/1
  HostRTI/1 -> MUX_DacI/1
  tx_source_select/1 -> MUX_DacI/2, MUX_DacQ/2
  REP_TxI/1 -> MUX_DacI/3
  HostRTQ/1 -> MUX_DacQ/1
  REP_TxQ/1 -> MUX_DacQ/3
  MUX_DacI/1 -> tx_dataOutI/1
  MUX_DacQ/1 -> tx_dataOutQ/1
  REP_TxValid/1 -> T_repValid/1
  RxValidConst/1 -> MUX_RxValid/1
  adc_dataInI/1 -> AdcCapI/1
  AdcCapI/1 -> AdcRTI/1
  AdcRTI/1 -> AdcStabI/1
  AdcStabI/1 -> MUX_RxI/1
  adc_dataInQ/1 -> AdcCapQ/1
  AdcCapQ/1 -> AdcRTQ/1
  AdcRTQ/1 -> AdcStabQ/1
  AdcStabQ/1 -> MUX_RxQ/1
  Receiver/10(cnt_descr_in) -> cnt_descr_in/1
  Receiver/11(cnt_frame_start) -> cnt_frame_start/1
  Receiver/12(cnt_vit_reset) -> cnt_vit_reset/1
  Receiver/13(cnt_deint_valid) -> cnt_deint_valid/1
  Receiver/14(cnt_dec_bits) -> cnt_dec_bits/1
  Receiver/15(cnt_bist_start) -> cnt_bist_start/1
  DbgSentinelConst/1 -> dbg_sentinel/1
  skip_count/1 -> Receiver/6(skip_count)
  Receiver/16(cap_in) -> cap_in/1
  Receiver/17(cap_deint) -> cap_deint/1
  Receiver/18(cap_out) -> cap_out/1
  Receiver/19(cap_cad) -> cap_cad/1
  Receiver/20(rstcs_count) -> rstcs_count/1, FrameStatProbe/2(rstcsCnt)
  Receiver/21(cfc_est) -> cfc_est/1, FsCfcSi/1
  Receiver/5(debugI) -> debugI/1
  Receiver/6(debugQ) -> debugQ/1
  Transmitter/9(extWordPop) -> PopRT/1
  PopRT/1 -> PopDly/1, PopEdge/1
  PopDly/1 -> PopEdge/2
  byte_data/1 -> ByteWordBuffer/1(dataIn)
  byte_valid/1 -> ByteWordBuffer/2(validIn)
  PopEdge/1 -> ByteWordBuffer/3(popReq)
  byte_first/1 -> ByteWordBuffer/4(firstIn)
  ByteWordBuffer/3(readyNext) -> ReadyDly/1
  ReadyDly/1 -> byte_ready/1
  ByteWordBuffer/1(word) -> WordRT/1
  ByteWordBuffer/2(avail) -> AvailRT/1
  ByteWordBuffer/4(wordFirst) -> FirstRT/1
  WordRT/1 -> Transmitter/5(extWord)
  AvailRT/1 -> Transmitter/6(extWordAvail)
  FirstRT/1 -> Transmitter/8(extWordFirst)
  tx_data_source/1 -> ByteSel/1
  ByteSel/1 -> SelRT/1
  SelRT/1 -> Transmitter/7(extBitSel)
  byte_rx_ready/1 -> RxReadyRT/1, ByteRxFifo/5(ready), FrameStatWordCnt/2(rdy)
  Receiver/22(recBit) -> ByteSerializer/1(bitIn)
  Receiver/23(recBitValid) -> ByteSerializer/2(bitValid)
  Receiver/24(recStart) -> ByteSerializer/3(start), FrameStatChecksum/3(strobe), FrameStatProbe/7(strobe)
  RxReadyRT/1 -> ByteSerializer/4(ready)
  ByteSerializer/1(word) -> SerWordRT/1, FrameStatChecksum/1(word)
  ByteSerializer/2(wordTog) -> SerTogRT/1, FrameStatChecksum/2(wordTog)
  ByteSerializer/3(wordLast) -> SerLastRT/1
  ByteSerializer/4(wordFirst) -> SerFirstRT/1
  SerWordRT/1 -> ByteRxFifo/1(word)
  SerTogRT/1 -> ByteRxFifo/2(tog)
  SerLastRT/1 -> ByteRxFifo/3(wLast)
  SerFirstRT/1 -> ByteRxFifo/4(wFirst)
  ByteRxFifo/1(outWord) -> byte_rx_data/1
  ByteRxFifo/2(valid) -> byte_rx_valid/1, FrameStatWordCnt/1(vld)
  ByteRxFifo/3(outLast) -> byte_rx_last/1
  ByteRxFifo/4(outFirst) -> byte_rx_user/1
  ByteRxFifo/5(ovf) -> byte_fifo_ovf/1
  cs_prop_gain/1 -> Receiver/7(cs_prop_gain)
  cs_integ_gain/1 -> Receiver/8(cs_integ_gain)
  ss_prop_gain/1 -> Receiver/9(ss_prop_gain)
  ss_integ_gain/1 -> Receiver/10(ss_integ_gain)
  agc_loop_gain/1 -> Receiver/11(agc_loop_gain)
  cfo_threshold/1 -> Receiver/12(cfo_threshold)
  Receiver/25(fs_runmax) -> FsRunSi/1
  FsRunSi/1 -> FrameStatProbe/3(runMax)
  FsAgcZero/1 -> FrameStatProbe/4(adcFor)
  FsCfcSi/1 -> FrameStatProbe/5(cfcEst)
  FrameStatChecksum/1(chk) -> FrameStatProbe/6(chk)
  FrameStatProbe/1(rec) -> FrameStatFifo/1(rec)
  FrameStatProbe/2(push) -> FrameStatFifo/2(push)
  framestat_pop/1 -> FrameStatFifo/3(popTok)
  FrameStatFifo/1(headLo) -> framestat_head_lo/1
  FrameStatFifo/2(headHi) -> framestat_head_hi/1
  FrameStatFifo/3(stat) -> framestat_stat/1
  FrameStatWordCnt/1(cnt) -> framestat_wordcnt/1

== system commhdlQPSKTxRxLoopback/Capture Tx Diagnostics/Subsystem ==
  In1 : Inport
  Enable : EnablePort
  To Workspace : ToWorkspace  VariableName=simQPSKSym  SampleTime=-1
      settings: Save2DSignal=2-D array (concatenate along first dimension)
  wires:
  In1/1 -> To Workspace/1

== system commhdlQPSKTxRxLoopback/Capture Tx Diagnostics/Subsystem1 ==
  In1 : Inport
  Enable : EnablePort
  To Workspace1 : ToWorkspace  VariableName=simTxWaveform  SampleTime=-1
      settings: Save2DSignal=2-D array (concatenate along first dimension)
  wires:
  In1/1 -> To Workspace1/1

== system commhdlQPSKTxRxLoopback/Channel/Mod 1 ==
  In1 : Inport
  Constant : Constant  SampleTime=-1
  Mod : Math  Operator=mod
  Out1 : Outport
  wires:
  Mod/1 -> Out1/1
  In1/1 -> Mod/1
  Constant/1 -> Mod/2

== system commhdlQPSKTxRxLoopback/Receiver/Capture Data Bits ==
  dataOut : Inport
  dataSrt : Inport  Port=2
  dataEnd : Inport  Port=3
  valid : Inport  Port=4
  Display : Display
  Display1 : Display
  Display2 : Display
  MATLAB Function : MATLAB Function  TreatAsAtomicUnit=on
  To Workspace : ToWorkspace  VariableName=RxOut  SampleTime=-1
      settings: Save2DSignal=2-D array (concatenate along first dimension)
  To Workspace1 : ToWorkspace  VariableName=RxOutSrt  SampleTime=-1
      settings: Save2DSignal=2-D array (concatenate along first dimension)
  To Workspace2 : ToWorkspace  VariableName=RxOutEnd  SampleTime=-1
      settings: Save2DSignal=2-D array (concatenate along first dimension)
  count_out : Outport
  packets_out : Outport  Port=2
  bit_errors_out : Outport  Port=3
  wires:
  dataOut/1 -> MATLAB Function/2(datain), To Workspace/1
  dataSrt/1 -> MATLAB Function/3(start), To Workspace1/1
  dataEnd/1 -> MATLAB Function/4(stop), To Workspace2/1
  valid/1 -> MATLAB Function/1(valid)
  MATLAB Function/1(count_out) -> count_out/1, Display/1
  MATLAB Function/2(packets_out) -> packets_out/1, Display1/1
  MATLAB Function/3(bit_errors_out) -> bit_errors_out/1, Display2/1

== system commhdlQPSKTxRxLoopback/Receiver/QPSK Rx ==
  dataIn : Inport  OutDataTypeStr=fixdt(1,16,14)  PortDimensions=1  SampleTime=1/(Rsym*SamplesPerSymbol)
      settings: SignalType=complex
  validIn : Inport  Port=2  OutDataTypeStr=boolean  PortDimensions=1  SampleTime=1/(Rsym*SamplesPerSymbol)
  rstCS : Inport  Port=3  OutDataTypeStr=boolean  PortDimensions=1
      settings: SignalType=complex
  debugMuxCtrl : Inport  Port=4  OutDataTypeStr=uint32  PortDimensions=1  SampleTime=1/(Rsym*SamplesPerSymbol)
  Automatic Gain Control : Subsystem  mask{Ref=AGCReference, LFG=AGCLoopGain}
      mask prompts: Ref "Error Detector Reference:"; LFG "Loop Filter Gain"
  Bus Creator : BusCreator  Inputs=4
  Bus Creator1 : BusCreator  Inputs=3
  Complex to Real-Imag : ComplexToRealImag
  Constant : Constant  Value=true  SampleTime=1/(Rsym*SamplesPerSymbol)
  Data Type Conversion : DataTypeConversion  OutDataTypeStr=int16  ConvertRealWorld=Stored Integer (SI)  SaturateOnIntegerOverflow=off  RndMeth=Floor
  Delay{,1..8} (9 alike) : Delay  DelayLength=1
  Frequency and Time Synchronizer : Subsystem
      settings: PortSchema="{\"entries\":[{\"content\":{\"sides\":[{\"content\":{\"connectorIds\":[\"In1\",\"In2\"]},\"type\":\"ConnectorPlacement.EquallySpacedRectSide\",\"uuid\":\"8bc6a452-5111-4806-8ca9-335cb622aea6\"},{\"content\":{\"connectorIds\":[\"Out1\",\"Out2\",\"Out3\",\"Out4\"],\"side\":\"RIGHT\"},\"type\":\"ConnectorPlacement.EquallySpacedRectSide\",\"uuid\":\"b0f43c98-f5c0-4f62-94ae-d69789942eef\"},{\"content\":{\"connectorIds\":[\"In3\",\"Out7\",\"Out8\"],\"side\":\"TOP\"},\"type\":\"ConnectorPlacement.EquallySpacedRectSide\",\"uuid\":\"427ff3b3-b896-4008-9584-d311480df763\"},{\"content\":{\"connectorIds\":[\"Out5\",\"Out6\"],\"side\":\"BOTTOM\"},\"type\":\"ConnectorPlacement.EquallySpacedRectSide\",\"uuid\":\"f704cb90-80a1-4198-8b72-e70182b45e73\"},{\"content\":{\"side\":\"HIDDEN\"},\"type\":\"ConnectorPlacement.EquallySpacedRectSide\",\"uuid\":\"f6309498-1e43-486f-b6b5-2c6570711f8e\"}]},\"type\":\"ConnectorPlacement.EquallySpacedConnector\",\"uuid\":\"f0ce492e-c9e1-4b35-98ef-84d77b696cfe\"}],\"packageUris\":[\"http://schema.mathworks.com/mf0/Connector/R2020b\"],\"version\":\"1.0\"}"
  HDL Data Descrambler : Subsystem
  Index Vector : MultiPortSwitch  DataPortOrder=Zero-based contiguous  Inputs=4  DiagnosticForDefault=None  zeroidx=on  SaturateOnIntegerOverflow=off  InputSameDT=off
  QPSK Demodulator : Subsystem
  RRC Receive Filter : dsphdlfiltering2/Discrete FIR Filter  NumeratorSource=Property  Numerator=RRCCoef  NumeratorPrototype=[]  FilterStructure=Direct form systolic  SerializationOption=Minimum number of cycles between valid input samples  NumCycles=2  NumberOfMultipliers=2  SimulateUsing=Code generation  roundingMode=Floor  overflowMode=off  CoefficientsDataTypeStr=Inherit: Same word length as input  OutputDataTypeStr=Inherit: Same word length as input  ResetInputPort=off  HDLGlobalReset=off  CoeffMultiplier=Multiplier  UseMultForPow2Coeff=on  FrameInputSymmOptim=off
  dataOut : Outport
  ctrlOut : Outport  Port=2
  rxDiagBus : Outport  Port=3
  debugIOut : Outport  Port=4
  debugQOut : Outport  Port=5
  debugValid : Outport  Port=6
  wires:
  rstCS/1 -> Frequency and Time Synchronizer/3(rstCS)
  QPSK Demodulator/1(dataOut) -> HDL Data Descrambler/1(dataIn)
  validIn/1 -> Automatic Gain Control/2(validIn)
  Automatic Gain Control/2(validOut) -> RRC Receive Filter/2
  RRC Receive Filter/1 -> Frequency and Time Synchronizer/1(dataIn)
  HDL Data Descrambler/3(endOut) -> Bus Creator1/2  "endOut"
  QPSK Demodulator/3(endOut) -> HDL Data Descrambler/3(endIn)
  Frequency and Time Synchronizer/8(normCoarseFreqEst) -> Bus Creator/2  "normCoarseFreqEst"
  Bus Creator1/1 -> ctrlOut/1
  HDL Data Descrambler/2(startOut) -> Bus Creator1/1  "startOut"
  Frequency and Time Synchronizer/3(endOut) -> QPSK Demodulator/3(endIn)
  RRC Receive Filter/2 -> Frequency and Time Synchronizer/2(validIn)
  Frequency and Time Synchronizer/7(nSynced) -> Bus Creator/1  "nSynced"
  Bus Creator/1 -> Delay/1
  Automatic Gain Control/1(dataOut) -> Delay1/1, RRC Receive Filter/1
  Frequency and Time Synchronizer/1(dataOut) -> Delay4/1, QPSK Demodulator/1(dataIn), Bus Creator/3  "QPSKConstellationPoints"
  dataIn/1 -> Automatic Gain Control/1(dataIn)
  HDL Data Descrambler/1(dataOut) -> dataOut/1
  HDL Data Descrambler/4(validOut) -> Bus Creator1/3  "validOut"
  QPSK Demodulator/2(startOut) -> HDL Data Descrambler/2(startIn)
  Frequency and Time Synchronizer/2(startOut) -> QPSK Demodulator/2(startIn)
  Frequency and Time Synchronizer/4(validOut) -> QPSK Demodulator/4(validIn), Bus Creator/4  "QPSKConstellationValid"
  QPSK Demodulator/4(validOut) -> HDL Data Descrambler/4(validIn)
  Delay/1 -> rxDiagBus/1
  Frequency and Time Synchronizer/5(postSymbolSync) -> Delay2/1
  Frequency and Time Synchronizer/6(postCarrierSync) -> Delay3/1
  debugMuxCtrl/1 -> Index Vector/1
  Complex to Real-Imag/2 -> debugQOut/1
  Complex to Real-Imag/1 -> debugIOut/1
  Data Type Conversion/1 -> Delay6/1
  Delay1/1 -> Index Vector/2
  Delay2/1 -> Index Vector/3
  Delay3/1 -> Index Vector/4
  Delay4/1 -> Index Vector/5
  Delay5/1 -> Data Type Conversion/1
  Index Vector/1 -> Delay5/1
  Delay6/1 -> Complex to Real-Imag/1
  Delay7/1 -> debugValid/1
  Delay8/1 -> Delay7/1
  Constant/1 -> Delay8/1

== system commhdlQPSKTxRxLoopback/Transmitter/Input Data ==
  enb : Inport
  reset : Inport  Port=2
  Cast To Boolean : DataTypeConversion  OutDataTypeStr=boolean  SaturateOnIntegerOverflow=off  RndMeth=Floor
  Delay : Delay  DelayLength=1
  Display : Display
  Message Generator : Subsystem
  Terminator : Terminator
  Terminator1 : Terminator
  txData : Outport
  txValid : Outport  Port=2
  msg_count_out : Outport  Port=3
  wires:
  Message Generator/4(valid) -> txValid/1
  Message Generator/1(out) -> txData/1
  enb/1 -> Message Generator/2(enable)
  Message Generator/5(count) -> Display/1
  Message Generator/2(stop) -> Delay/1
  Delay/1 -> Cast To Boolean/1
  Cast To Boolean/1 -> Message Generator/1(reset)
  reset/1 -> Terminator/1
  Message Generator/3(start) -> Terminator1/1
  Message Generator/6(msg_count_out) -> msg_count_out/1

== system commhdlQPSKTxRxLoopback/Transmitter/QPSK Tx ==
  dataIn : Inport  OutDataTypeStr=boolean  PortDimensions=1
  validIn : Inport  Port=2  OutDataTypeStr=boolean  PortDimensions=1
  Bit Packetizer : Subsystem
  Bus Creator : BusCreator  Inputs=2
  HDL Data Scrambler : Subsystem
  QPSK Modulator : Subsystem
  RRC Transmit Filter : Subsystem
  dataReady : Outport
  dataOut : Outport  Port=2
  txDiagBus : Outport  Port=3
  validOut : Outport  Port=4
  wires:
  validIn/1 -> Bit Packetizer/2(validIn)
  RRC Transmit Filter/2(validOut) -> validOut/1
  HDL Data Scrambler/1(dataOut) -> QPSK Modulator/1(dataIn)
  Bit Packetizer/1(bitsOut) -> HDL Data Scrambler/1(dataIn)
  QPSK Modulator/2(validOut) -> Bus Creator/2, RRC Transmit Filter/2(validIn)  "QPSKConstellationValid"
  dataIn/1 -> Bit Packetizer/1(dataIn)
  Bit Packetizer/3(dataEnd) -> HDL Data Scrambler/3(endIn)
  HDL Data Scrambler/2(validOut) -> QPSK Modulator/2(validIn)
  RRC Transmit Filter/1(dataOut) -> dataOut/1
  QPSK Modulator/1(dataOut) -> Bus Creator/1, RRC Transmit Filter/1(dataIn)  "QPSKConstellationPoints"
  Bit Packetizer/2(dataStart) -> HDL Data Scrambler/2(startIn)
  Bit Packetizer/5(dataReady) -> dataReady/1
  Bus Creator/1 -> txDiagBus/1
  Bit Packetizer/4(bitsValid) -> HDL Data Scrambler/4(validIn)
